simulink model "avlmath"  (R2025a)
settings: Solver=VariableStepAuto  StartTime=0.0  StopTime=2.0  RelTol=1e-3
settings Model: Creator=sanjay  LastModifiedBy=sanjay

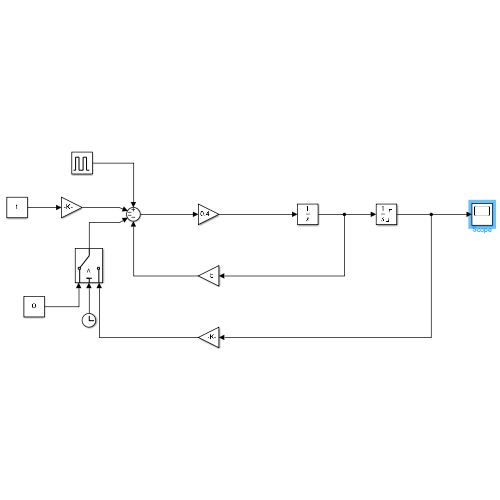
[thumbnail: Simulink's stored preview of the top-level diagram]
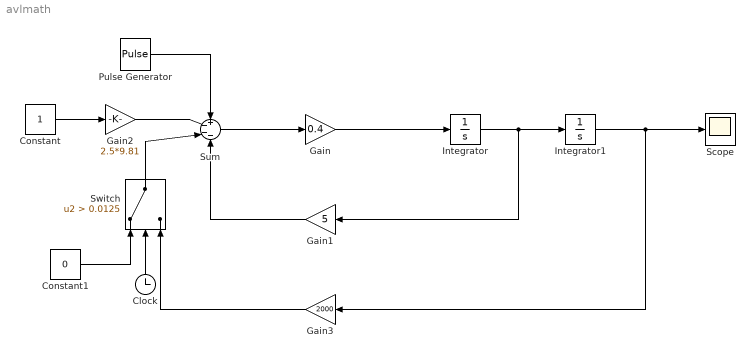
== system avlmath ==
  Clock : Clock
  Constant : Constant
  Constant1 : Constant  Value=0
  Gain : Gain  Gain=0.4
  Gain1 : Gain  Gain=5
  Gain2 : Gain  Gain=2.5*9.81
  Gain3 : Gain  Gain=2000
  Integrator : Integrator
  Integrator1 : Integrator  LimitOutput=on  LowerSaturationLimit=0
  Pulse Generator : DiscretePulseGenerator  PulseType=Time based  Amplitude=900  PulseWidth=0.625
  Scope : Scope
      settings: ActiveDisplayYMinimum=-0.10080746550371689  ActiveDisplayYMaximum=1.2598419610872376
  Sum : Sum  Inputs=+---
  Switch : Switch  Criteria=u2 > Threshold  Threshold=0.0125  SaturateOnIntegerOverflow=off  InputSameDT=off
  wires:
  Pulse Generator/1 -> Sum/1
  Constant/1 -> Gain2/1
  Gain2/1 -> Sum/2
  Sum/1 -> Gain/1
  Gain/1 -> Integrator/1
  Integrator/1 -> Gain1/1, Integrator1/1
  Integrator1/1 -> Gain3/1, Scope/1
  Gain1/1 -> Sum/4
  Switch/1 -> Sum/3
  Gain3/1 -> Switch/3
  Clock/1 -> Switch/2
  Constant1/1 -> Switch/1
